simulink model "hopper_6dof_NED_v2_ctv"  (R2025b)
settings: Solver=FixedStepAuto  StartTime=0.0  StopTime=30  FixedStep=1e-3  RelTol=1e-5
values from neighbouring files (symbols this model uses):
  ENGINE = size_engine(IN)    [main_ctv.m]
  fu_mass_profile = linspace(0.1, IN.propulsion.fuel_mass, 200)    [generateBaffleLUT_ctv.m]
  fu_mdot_data = mdot_data(:,2)    [load_lookup_ctv.m]
  g = p.g    [HopperLinearization_6DOF_inertial.m]
  IN = mission_inputs()    [main_ctv.m]
  K1flat = zeros(length(tgrid),52)    [LinerizationMaster_ctv.m]
  K2grid = GainTable.K2'    [LinerizationMaster_ctv.m]
  OUT = Outputs(IN, VEH, TANKS, STRUCT)    [main_ctv.m]
  ox_mass_profile = linspace(0.1, IN.propulsion.oxidizer_mass, 200)    [generateBaffleLUT_ctv.m]
  ox_mdot_data = mdot_data(:,3)    [load_lookup_ctv.m]
  r_leg_1 = [0 IN.legs.feet_radial_dist 0]    [main_ctv.m]
  r_leg_2 = [0 -IN.legs.feet_radial_dist 0]    [main_ctv.m]
  r_leg_3 = [0 0 IN.legs.feet_radial_dist ]    [main_ctv.m]
  r_leg_4 = [0 0 -IN.legs.feet_radial_dist]    [main_ctv.m]
  tank_r = TANKS.singular.radius    [generateBaffleLUT_ctv.m]
  TANKS = size_tanks(IN)    [main_ctv.m]
  Target_Trajectory = [x_trajectory;y_trajectory;z_trajectory;    vx_trajectory;vy_trajectory; vz_trajectory;    P_trajectory; Q_trajectory; R_trajectory ... (first row only)    [LinerizationMaster_ctv.m]
  tgrid = t    [LinerizationMaster_ctv.m]
  thrust_data = mdot_data(:,1)    [load_lookup_ctv.m]
  unom = [T_profile, delta_y_profile, delta_z_profile, rcsp]    [LinerizationMaster_ctv.m]
undefined symbols (not defined in the file or in its folder): cg_init, dcg_dMfu_table, dcg_dMox_table, dI_dMfu_table, dI_dMox_table, engine_cg, engine_mass, fu_axial_damping_ratios, fu_lateral_damping_ratios, fu_masses, MoI_init, mount_cg, ox_axial_damping_ratios, ox_lateral_damping_ratios, ox_masses, pressureLevels, uwndTable, VEH, vwndTable
libraries: fl_lib x31, nesl_utility x25, matrix_library x18, SimscapeFluids_lib x10, simulink_extras x7, slpidlib x7, simulink x7, dspindex x3, aerolibanim x1, commrandsrc3 x1, aerolibutil x1, dspsrcs4 x1
(part 2 of 7)

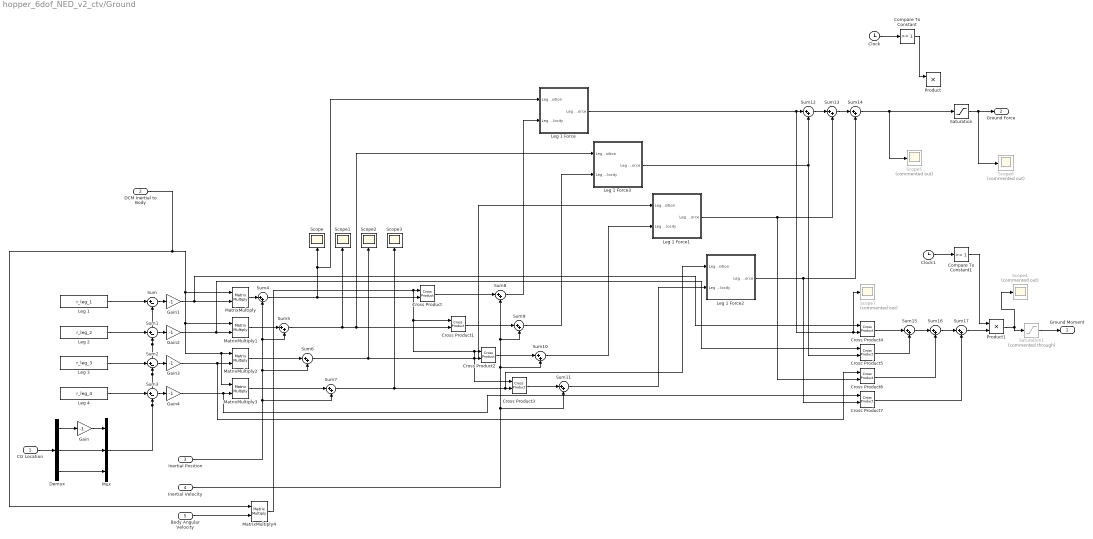
== system hopper_6dof_NED_v2_ctv/Ground  ==
  CG Location : Inport
  DCM Inertial to Body : Inport  Port=2
  Inertial Position : Inport  Port=3
  Inertial Velocity : Inport  Port=4
  Body Angular Velocity : Inport  Port=5
  Clock : Clock
  Clock1 : Clock
  Compare To Constant : simulink/Logic and Bit Operations/Compare To Constant  relop=>=  const=1  OutDataTypeStr=boolean
  Compare To Constant1 : simulink/Logic and Bit Operations/Compare To Constant  relop=>=  const=1  OutDataTypeStr=boolean
  Cross Product{,1..7} (8 alike) : matrix_library/Cross Product
  Demux : Demux  Outputs=3
  Gain{,1..4} (5 alike) : Gain  Gain=-1
  Leg 1 : Constant  Value=r_leg_1
  Leg 1 Force : Subsystem
  Leg 1 Force1 : Subsystem
  Leg 1 Force2 : Subsystem
  Leg 1 Force3 : Subsystem
  Leg 2 : Constant  Value=r_leg_2
  Leg 3 : Constant  Value=r_leg_3
  Leg 4 : Constant  Value=r_leg_4
  MatrixMultiply{,1..4} (5 alike) : Product  Multiplication=Matrix(*)
  Mux : Mux  Inputs=3
  Product : Product
  Product1 : Product
  Saturation : Saturate  UpperLimit=inf  LowerLimit=0
  Saturation1 : Saturate  Commented=through  UpperLimit=inf  LowerLimit=0
  Scope{,1..3} (4 alike) : Scope
      Scope settings: ActiveDisplayYMinimum=-19.811154048207108  ActiveDisplayYMaximum=167.31101950999761  DataLoggingVariableName=ScopeData24
      Scope1 settings: ActiveDisplayYMinimum=182.10765195211306  ActiveDisplayYMaximum=183.93696889205802  DataLoggingVariableName=ScopeData30
      Scope2 settings: DataLoggingVariableName=ScopeData31
      Scope3 settings: DataLoggingVariableName=ScopeData42
  Scope{4..7} (4 alike) : Scope  Commented=on
      Scope4 settings: ActiveDisplayYMinimum=-3.0293963365637429E+7  ActiveDisplayYMaximum=2.2731893212350109E+8  DataLoggingVariableName=ScopeData43
      Scope5 settings: ActiveDisplayYMinimum=-31343.151613259419  ActiveDisplayYMaximum=282088.36451933486  DataLoggingVariableName=ScopeData44
      Scope6 settings: ActiveDisplayYMinimum=-136.62925150266653  ActiveDisplayYMaximum=1229.6632635239991  DataLoggingVariableName=ScopeData45
      Scope7 settings: ActiveDisplayYMinimum=-3.5823523450793636E+8  ActiveDisplayYMaximum=5.8466661508525646E+8  DataLoggingVariableName=ScopeData61
  Sum{,1..3} (4 alike) : Sum  Inputs=|+-
  Sum{4..17} (14 alike) : Sum  Inputs=|++
  Ground Moment : Outport
  Ground Force : Outport  Port=2
  wires:
  Demux/2 -> Mux/2
  Demux/3 -> Mux/3
  Leg 1/1 -> Sum/1
  Leg 2/1 -> Sum1/1
  Leg 3/1 -> Sum2/1
  Leg 4/1 -> Sum3/1
  Mux/1 -> Sum3/2, Sum1/2, Sum/2, Sum2/2
  Sum/1 -> Gain1/1
  DCM Inertial to Body/1 -> MatrixMultiply4/1, MatrixMultiply1/1, MatrixMultiply3/1, MatrixMultiply2/1, MatrixMultiply/1
  Sum1/1 -> Gain2/1
  Sum2/1 -> Gain3/1
  Sum3/1 -> Gain4/1
  MatrixMultiply3/1 -> Sum7/1
  MatrixMultiply2/1 -> Sum6/1
  MatrixMultiply1/1 -> Sum5/1
  MatrixMultiply/1 -> Sum4/1
  Inertial Position/1 -> Sum7/2, Sum6/2, Sum5/2, Sum4/2
  Sum4/1 -> Scope/1, Leg 1 Force/1(Leg Position), Cross Product/2
  Sum5/1 -> Leg 1 Force3/1(Leg Position), Cross Product1/2, Scope1/1
  Sum6/1 -> Leg 1 Force1/1(Leg Position), Cross Product2/2, Scope2/1
  Sum7/1 -> Leg 1 Force2/1(Leg Position), Cross Product3/2, Scope3/1
  Body Angular Velocity/1 -> MatrixMultiply4/2
  MatrixMultiply4/1 -> Cross Product1/1, Cross Product3/1, Cross Product2/1, Cross Product/1
  Cross Product/1 -> Sum8/1
  Cross Product1/1 -> Sum9/1
  Cross Product2/1 -> Sum10/1
  Cross Product3/1 -> Sum11/1
  Inertial Velocity/1 -> Sum11/2, Sum10/2, Sum9/2, Sum8/2
  Leg 1 Force/1(Leg 1 Force) -> Scope7/1, Cross Product4/2, Sum12/1
  Leg 1 Force3/1(Leg 1 Force) -> Cross Product5/2, Sum12/2
  Sum12/1 -> Sum13/1
  Leg 1 Force1/1(Leg 1 Force) -> Cross Product6/2, Sum13/2
  Sum13/1 -> Sum14/1
  Leg 1 Force2/1(Leg 1 Force) -> Cross Product7/2, Sum14/2
  Cross Product4/1 -> Sum15/1
  Sum15/1 -> Sum16/1
  Cross Product5/1 -> Sum15/2
  Cross Product6/1 -> Sum16/2
  Sum16/1 -> Sum17/1
  Cross Product7/1 -> Sum17/2
  Sum8/1 -> Leg 1 Force/2(Leg Velocity)
  Sum9/1 -> Leg 1 Force3/2(Leg Velocity)
  Sum10/1 -> Leg 1 Force1/2(Leg Velocity)
  Sum11/1 -> Leg 1 Force2/2(Leg Velocity)
  Saturation/1 -> Ground Force/1, Scope6/1
  Saturation1/1 -> Ground Moment/1
  Gain/1 -> Mux/1
  Gain1/1 -> Cross Product4/1, MatrixMultiply/2
  Gain2/1 -> Cross Product5/1, MatrixMultiply1/2
  Gain3/1 -> Cross Product6/1, MatrixMultiply2/2
  Gain4/1 -> Cross Product7/1, MatrixMultiply3/2
  Sum14/1 -> Saturation/1, Scope5/1
  Clock1/1 -> Compare To Constant1/1
  Compare To Constant1/1 -> Product1/1
  Sum17/1 -> Product1/2
  Product1/1 -> Scope4/1, Saturation1/1
  CG Location/1 -> Demux/1
  Demux/1 -> Gain/1
  Clock/1 -> Compare To Constant/1
  Compare To Constant/1 -> Product/1

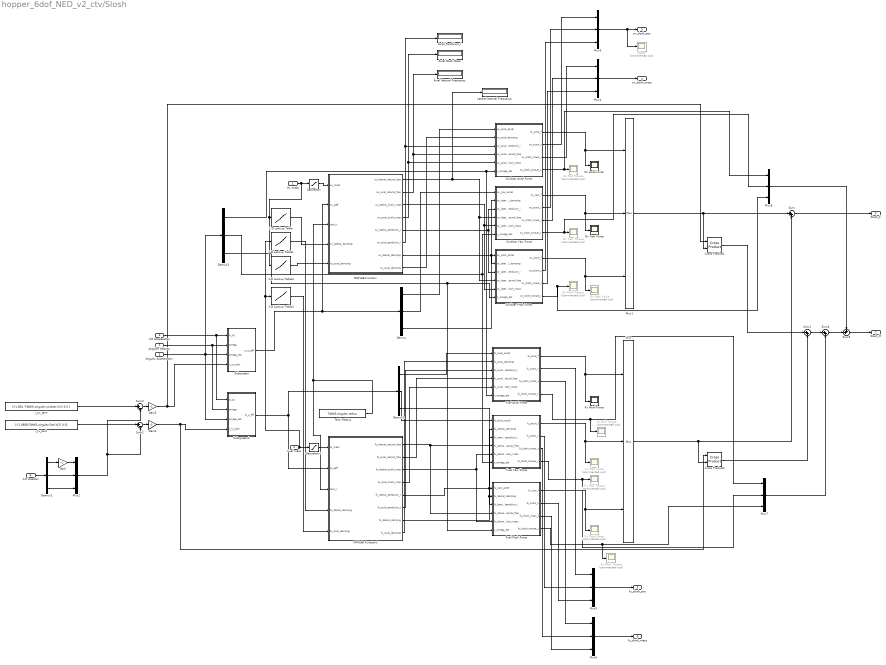
== system hopper_6dof_NED_v2_ctv/Slosh ==
  Ox mass : Inport
  Fuel mass : Inport  Port=2
  CG Acceleration : Inport  Port=3
  Angular Velocity : Inport  Port=4
  Angular Acceleration : Inport  Port=5
  CG Location : Inport  Port=6
  1-D Lookup Table : Lookup_n-D  NumberOfTableDimensions=1  BreakpointsForDimension1=ox_mass_profile  Table=ox_lateral_damping_ratios  InternalRulePriority=Speed  RndMeth=Simplest
  1-D Lookup Table1 : Lookup_n-D  NumberOfTableDimensions=1  BreakpointsForDimension1=fu_mass_profile  Table=fu_lateral_damping_ratios  InternalRulePriority=Speed  RndMeth=Simplest
  1-D Lookup Table2 : Lookup_n-D  NumberOfTableDimensions=1  BreakpointsForDimension1=fu_mass_profile  Table=fu_axial_damping_ratios  InternalRulePriority=Speed  RndMeth=Simplest
  1-D Lookup Table4 : Lookup_n-D  NumberOfTableDimensions=1  BreakpointsForDimension1=ox_mass_profile  Table=ox_axial_damping_ratios  InternalRulePriority=Speed  RndMeth=Simplest
  Axial Natural Frequency : Display
  Axial Slosh Mass : Display
  Axial_Pendulum_l : Display
  Cross Product1 : matrix_library/Cross Product
  Cross Product2 : matrix_library/Cross Product
  Demux{,1..3} (4 alike) : Demux  Outputs=3
  Fu Axial Force : Scope
      settings: ActiveDisplayYMinimum=-4.5487995330933861  ActiveDisplayYMaximum=10.430303988696288  DataLoggingVariableName=ScopeData38
  Fu Pitch Force : Scope  Commented=on
      settings: ActiveDisplayYMinimum=-2.9742058993087932  ActiveDisplayYMaximum=15.331760127930639  DataLoggingVariableName=ScopeData40
  Fu Pitch Torque : Scope  Commented=on
      settings: ActiveDisplayYMinimum=-0.19116574787256713  ActiveDisplayYMaximum=0.19970427620804132  DataLoggingVariableName=ScopeData87
  Fu Roll Torque : Scope  Commented=on
      settings: ActiveDisplayYMinimum=-9.5580450498277436  ActiveDisplayYMaximum=8.6061310713641461  DataLoggingVariableName=ScopeData86
  Fu Yaw Force : Scope  Commented=on
      settings: ActiveDisplayYMinimum=-1.96682346554972  ActiveDisplayYMaximum=2.7427386100438831  DataLoggingVariableName=ScopeData39
  Fu Yaw Torque : Scope  Commented=on
      settings: ActiveDisplayYMinimum=-3.6886267521568623  ActiveDisplayYMaximum=3.9647425854021145  DataLoggingVariableName=ScopeData82
  Fuel Axial Force : Subsystem
  Fuel Pitch Force : Subsystem
  Fuel Yaw Force : Subsystem
  Gain : Gain  Gain=-1
  Gain3 : Gain  Gain=-1
  Gain4 : Gain  Gain=-1
  Lateral Natural Frequency : Display
  MATLAB Function : MATLAB Function  TreatAsAtomicUnit=on
  MATLAB Function1 : MATLAB Function  TreatAsAtomicUnit=on
  Mux{,1..8} (9 alike) : Mux  Inputs=3
  Ox Axial Force : Scope
      settings: ActiveDisplayYMinimum=14.43010515330246  ActiveDisplayYMaximum=16.756383333748122  DataLoggingVariableName=ScopeData34
  Ox Pitch Force : Scope  Commented=on
      settings: ActiveDisplayYMinimum=-4.4950785008236629  ActiveDisplayYMaximum=22.001881619828325  DataLoggingVariableName=ScopeData36
  Ox Pitch Torque : Scope  Commented=on
      settings: ActiveDisplayYMinimum=-0.69593653498138675  ActiveDisplayYMaximum=0.79680864639954685  DataLoggingVariableName=ScopeData85
  Ox Roll Torque : Scope  Commented=on
      settings: ActiveDisplayYMinimum=-0.15656949128956149  ActiveDisplayYMaximum=0.79158034254760723  DataLoggingVariableName=ScopeData80
  Ox Yaw Force : Scope
      settings: ActiveDisplayYMinimum=-5.8284827308381395  ActiveDisplayYMaximum=24.723450598791928  DataLoggingVariableName=ScopeData37
  Ox Yaw Torque : Scope  Commented=on
      settings: ActiveDisplayYMinimum=-0.3482323750211066  ActiveDisplayYMaximum=0.31743853430357161  DataLoggingVariableName=ScopeData81
  Oxidizer Axial Force : Subsystem
  Oxidizer Pitch Force : Subsystem
  Oxidizer Yaw Force : Subsystem
  Saturation : Saturate  UpperLimit=inf  LowerLimit=0.01
  Saturation1 : Saturate  UpperLimit=inf  LowerLimit=0.01
  Scope : Scope  Commented=on
      settings: ActiveDisplayYMinimum=-0.0849364779794028  ActiveDisplayYMaximum=0.368207880424993  DataLoggingVariableName=ScopeData35
  Subsystem : Subsystem
  Subsystem1 : Subsystem
  Sum : Sum  Inputs=|++
  Sum1 : Sum  Inputs=|++
  Sum2 : Sum  Inputs=|+-
  Sum3 : Sum  Inputs=|+-
  Sum4 : Sum  Inputs=|++
  Sum5 : Sum  Inputs=++|
  Tank Radius : Constant  Value=TANKS.singular.radius  SampleTime=-1
  r_fu_tank : Constant  Value=[-(1.0668-TANKS.singular.fuel.h/2) 0 0]
  r_ox_tank : Constant  Value=[-(1.854 -TANKS.singular.oxidizer.h/2) 0 0 ]
  Slosh_F : Outport
  Slosh_M : Outport  Port=2
  ox_slosh_pos : Outport  Port=3
  ox_slosh_mass : Outport  Port=4
  fu_slosh_pos : Outport  Port=5
  fu_slosh_mass : Outport  Port=6
  wires:
  Ox mass/1 -> 1-D Lookup Table4/1, 1-D Lookup Table/1, Saturation/1
  CG Acceleration/1 -> Subsystem/1(a_cg), Subsystem1/1(a_cg)
  Angular Velocity/1 -> Subsystem/2(omega), Subsystem1/2(omega)
  Angular Acceleration/1 -> Subsystem/3(omega_dot), Subsystem1/3(omega_dot), Demux3/1
  Fuel mass/1 -> 1-D Lookup Table2/1, 1-D Lookup Table1/1, Saturation1/1
  Subsystem/1(ox_a_eff) -> Demux/1, MATLAB Function/2(ox_aeff)
  Subsystem1/1(fu_a_eff) -> Demux1/1, MATLAB Function1/2(fu_aeff)
  Demux/1 -> Oxidizer Axial Force/1(ox_axial_accel)
  Demux/2 -> Oxidizer Yaw Force/1(ox_yaw_accel)
  Demux/3 -> Oxidizer Pitch Force/1(ox_pitch_accel)
  Demux1/1 -> Fuel Axial Force/1(fu_axial_accel)
  Demux1/2 -> Fuel Yaw Force/1(fu_pitch_accel)
  Demux1/3 -> Fuel Pitch Force/1(fu_yaw_accel)
  MATLAB Function/1(ox_lateral_natural_freq) -> Lateral Natural Frequency/1, Oxidizer Pitch Force/4(ox_lateral_natural_freq), Oxidizer Yaw Force/4(ox_lateral_natural_freq)
  MATLAB Function/2(ox_axial_natural_freq) -> Axial Natural Frequency/1, Oxidizer Axial Force/4(ox_axial_natural_freq)
  MATLAB Function/3(ox_lateral_slosh_mass) -> Oxidizer Pitch Force/5(ox_lateral_slosh_mass), Oxidizer Yaw Force/5(ox_lateral_slosh_mass)
  MATLAB Function/4(ox_axial_slosh_mass) -> Axial Slosh Mass/1, Oxidizer Axial Force/5(ox_axial_slosh_mass)
  MATLAB Function/5(ox_lateral_pendulum_l) -> Oxidizer Yaw Force/3(ox_lateral_pendulum_l), Oxidizer Pitch Force/3(ox_lateral_pendulum_l)
  MATLAB Function/6(ox_axial_pendulum_l) -> Axial_Pendulum_l/1, Oxidizer Axial Force/3(ox_axial_pendulum_l)
  MATLAB Function/7(ox_lateral_damping) -> Oxidizer Yaw Force/2(ox_lateral_damping), Oxidizer Pitch Force/2(ox_lateral_damping)
  MATLAB Function/8(ox_axial_damping) -> Oxidizer Axial Force/2(ox_axial_damping)
  MATLAB Function1/1(fu_lateral_natural_freq) -> Fuel Pitch Force/4(fu_lateral_natural_freq), Fuel Yaw Force/4(fu_lateral_natural_freq)
  MATLAB Function1/2(fu_axial_natural_freq) -> Fuel Axial Force/4(fu_axial_natural_freq)
  MATLAB Function1/3(fu_lateral_slosh_mass) -> Fuel Yaw Force/5(fu_lateral_slosh_mass), Fuel Pitch Force/5(fu_lateral_slosh_mass)
  MATLAB Function1/4(fu_axial_slosh_mass) -> Fuel Axial Force/5(fu_axial_slosh_mass)
  MATLAB Function1/5(fu_lateral_pendulum_l) -> Fuel Yaw Force/3(fu_lateral_pendulum_l), Fuel Pitch Force/3(fu_lateral_pendulum_l)
  MATLAB Function1/6(fu_axial_pendulum_l) -> Fuel Axial Force/3(fu_axial_pendulum_l)
  MATLAB Function1/7(fu_lateral_damping) -> Fuel Yaw Force/2(fu_lateral_damping), Fuel Pitch Force/2(fu_lateral_damping)
  MATLAB Function1/8(fu_axial_damping) -> Fuel Axial Force/2(fu_axial_damping)
  Fuel Axial Force/1(fu_axial_f) -> Fu Axial Force/1, Mux/1
  Fuel Yaw Force/1(fu_pitch_f) -> Fu Yaw Force/1, Mux/2
  Oxidizer Axial Force/1(ox_axial_f) -> Ox Axial Force/1, Mux1/1
  Oxidizer Yaw Force/1(ox_yaw_f) -> Ox Yaw Force/1, Mux1/2
  Mux1/1 -> Cross Product1/2, Sum/1
  Mux/1 -> Sum/2, Cross Product2/2
  Sum/1 -> Slosh_F/1
  Cross Product1/1 -> Sum1/1
  Cross Product2/1 -> Sum1/2
  Tank Radius/1 -> MATLAB Function1/3(tank_r), MATLAB Function/3(tank_r)
  r_ox_tank/1 -> Sum3/1
  r_fu_tank/1 -> Sum2/1
  Mux2/1 -> Sum2/2, Sum3/2
  Sum3/1 -> Gain3/1
  Sum2/1 -> Gain4/1
  Fuel Pitch Force/1(fu_yaw_f) -> Mux/3, Fu Pitch Force/1
  Oxidizer Pitch Force/1(ox_pitch_f) -> Mux1/3, Ox Pitch Force/1
  Gain3/1 -> Cross Product1/1, Subsystem/4(r_ox_tank)
  Gain4/1 -> Cross Product2/1, Subsystem1/4(r_fu_tank)
  Demux2/3 -> Mux2/3
  CG Location/1 -> Demux2/1
  Demux2/2 -> Mux2/2
  Demux2/1 -> Gain/1
  Gain/1 -> Mux2/1
  Oxidizer Yaw Force/2(ox_slosh_y) -> Mux3/2
  Mux3/1 -> Scope/1, ox_slosh_pos/1
  Oxidizer Axial Force/3(ox_slosh_mass_x) -> Mux4/1
  Oxidizer Yaw Force/3(ox_slosh_mass_y) -> Mux4/2
  Oxidizer Pitch Force/2(ox_slosh_z) -> Mux3/3
  Oxidizer Pitch Force/3(ox_slosh_mass_z) -> Mux4/3
  Mux4/1 -> ox_slosh_mass/1
  Mux5/1 -> fu_slosh_pos/1
  Mux6/1 -> fu_slosh_mass/1
  Fuel Yaw Force/2(fu_slosh_y) -> Mux5/2
  Fuel Pitch Force/2(fu_slosh_z) -> Mux5/3
  Fuel Axial Force/3(fu_slosh_mass_x) -> Mux6/1
  Fuel Yaw Force/3(fu_slosh_mass_y) -> Mux6/2
  Fuel Pitch Force/3(fu_slosh_mass_z) -> Mux6/3
  Oxidizer Axial Force/2(ox_slosh_x) -> Mux3/1
  Fuel Axial Force/2(fu_slosh_x) -> Mux5/1
  Demux3/1 -> Oxidizer Axial Force/6(x_omega_dot), Fuel Axial Force/6(x_omega_dot)
  Demux3/2 -> Fuel Yaw Force/6(y_omega_dot), Oxidizer Yaw Force/6(y_omega_dot)
  Demux3/3 -> Fuel Pitch Force/6(z_omega_dot), Oxidizer Pitch Force/6(z_omega_dot)
  Fuel Axial Force/4(fu_slosh_torque_x) -> Mux7/1, Fu Roll Torque/1
  Fuel Yaw Force/4(fu_slosh_torque_y) -> Mux7/2, Fu Yaw Torque/1
  Fuel Pitch Force/4(fu_slosh_torque_z) -> Mux7/3, Fu Pitch Torque/1
  Oxidizer Axial Force/4(ox_slosh_torque_x) -> Mux8/1, Ox Roll Torque/1
  Oxidizer Pitch Force/4(ox_slosh_torque_z) -> Ox Pitch Torque/1, Mux8/3
  Sum1/1 -> Sum4/1
  Sum5/1 -> Slosh_M/1
  Sum4/1 -> Sum5/2
  Oxidizer Yaw Force/4(ox_slosh_torque_y) -> Mux8/2, Ox Yaw Torque/1
  Mux8/1 -> Sum5/1
  Mux7/1 -> Sum4/2
  Saturation/1 -> MATLAB Function/1(ox_mass)
  Saturation1/1 -> MATLAB Function1/1(fu_mass)
  1-D Lookup Table/1 -> MATLAB Function/4("ox_lateral_damping ")
  1-D Lookup Table1/1 -> MATLAB Function1/4("fu_lateral_damping ")
  1-D Lookup Table4/1 -> MATLAB Function/5("ox_axial_damping ")
  1-D Lookup Table2/1 -> MATLAB Function1/5("fu_axial_damping ")

== system hopper_6dof_NED_v2_ctv/Subsystem ==
  Thrust : Inport
  Fuel mdot : Lookup_n-D  NumberOfTableDimensions=1  BreakpointsForDimension1=thrust_data  Table=fu_mdot_data  InternalRulePriority=Speed  RndMeth=Simplest
  Ox mdot : Lookup_n-D  NumberOfTableDimensions=1  BreakpointsForDimension1=thrust_data  Table=ox_mdot_data  InternalRulePriority=Speed  RndMeth=Simplest
  Fu_mdot : Outport
  Ox_mdot : Outport  Port=2
  wires:
  Thrust/1 -> Ox mdot/1, Fuel mdot/1
  Fuel mdot/1 -> Fu_mdot/1
  Ox mdot/1 -> Ox_mdot/1

== system hopper_6dof_NED_v2_ctv/Subsystem1 ==
  Ox_mdot : Inport
  Fu_mdot : Inport  Port=2
  Integrator : Integrator
  Integrator1 : Integrator
  Ox Mass1 : Constant  Value=IN.propulsion.oxidizer_mass
  Ox Mass2 : Constant  Value=IN.propulsion.fuel_mass
  Saturation : Saturate  UpperLimit=IN.propulsion.oxidizer_mass  LowerLimit=0
  Saturation1 : Saturate  UpperLimit=IN.propulsion.fuel_mass  LowerLimit=0
  Sum : Sum  Inputs=|-+
  Sum1 : Sum  Inputs=|-+
  Ox Mass : Outport
  Fuel Mass : Outport  Port=2
  wires:
  Ox_mdot/1 -> Integrator/1
  Integrator/1 -> Sum/1
  Ox Mass1/1 -> Sum/2
  Sum/1 -> Saturation/1
  Saturation/1 -> Ox Mass/1
  Sum1/1 -> Saturation1/1
  Saturation1/1 -> Fuel Mass/1
  Fu_mdot/1 -> Integrator1/1
  Ox Mass2/1 -> Sum1/2
  Integrator1/1 -> Sum1/1

== system hopper_6dof_NED_v2_ctv/Subsystem2 ==
  Thrust : Inport
  Ox mass : Inport  Port=2
  Fu mass : Inport  Port=3
  If : If  NumInputs=2  IfExpression=u1 > 0 & u2 > 0
  If Action Subsystem : Subsystem  TreatAsAtomicUnit=on
  If Action Subsystem1 : Subsystem  TreatAsAtomicUnit=on
  Merge : Merge
  "Thrust " : Outport
  wires:
  Ox mass/1 -> If/1
  Fu mass/1 -> If/2
  If/1 -> If Action Subsystem/Action
  If/2 -> If Action Subsystem1/Action
  Thrust/1 -> If Action Subsystem1/1(Thrust), If Action Subsystem/1(Thrust)
  If Action Subsystem/1(Out1) -> Merge/1
  If Action Subsystem1/1(Out1) -> Merge/2
  Merge/1 -> "Thrust "/1

== system hopper_6dof_NED_v2_ctv/Subsystem3 ==
  Z : Inport
  W : Inport  Port=2
  Clock : Clock
  Compare To Constant : simulink/Logic and Bit Operations/Compare To Constant  relop=>=  const=5  OutDataTypeStr=boolean
  Constant : Constant
  If : If  NumInputs=2  IfExpression=u1 > -1e-3 & u2 > 0
  If Action Subsystem : Subsystem  TreatAsAtomicUnit=on
  Product : Product
  wires:
  Z/1 -> If/1
  W/1 -> If/2
  If/1 -> If Action Subsystem/Action
  Clock/1 -> Compare To Constant/1
  Compare To Constant/1 -> Product/2
  Constant/1 -> Product/1
  Product/1 -> If Action Subsystem/1(In1)

== system hopper_6dof_NED_v2_ctv/Subsystem4 ==
  Thrust : Inport
  Position : Inport  Port=2
  Velocity : Inport  Port=3
  Demux : Demux  Outputs=3
  Demux1 : Demux  Outputs=3
  If : If  NumInputs=2  IfExpression=u1 > -0.05 & u2 > 0
  If Action Subsystem : Subsystem  TreatAsAtomicUnit=on
  If Action Subsystem1 : Subsystem  TreatAsAtomicUnit=on
  Merge : Merge
  "Thrust " : Outport
  wires:
  If Action Subsystem1/1(Out1) -> Merge/2
  Merge/1 -> "Thrust "/1
  If Action Subsystem/1(Out1) -> Merge/1
  Thrust/1 -> If Action Subsystem1/1(Thrust), If Action Subsystem/1(Thrust)
  Position/1 -> Demux/1
  Demux1/3 -> If/2
  Demux/3 -> If/1
  If/1 -> If Action Subsystem1/Action
  If/2 -> If Action Subsystem/Action
  Velocity/1 -> Demux1/1

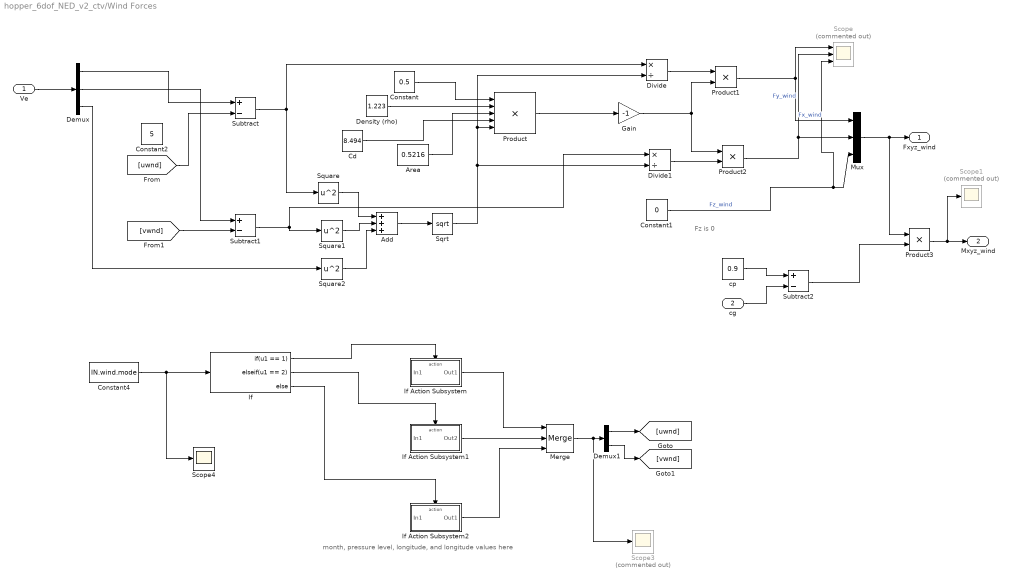
== system hopper_6dof_NED_v2_ctv/Wind Forces ==
  note: month, pressure level, longitude, and longitude values here
  note: Fz is 0
  Ve : Inport
  cg : Inport  Port=2
  Add : Sum  Inputs=+++
  Area : Constant  Value=0.5216
  Cd : Constant  Value=8.494
  Constant : Constant  Value=0.5
  Constant1 : Constant  Value=0
  Constant2 : Constant  Value=5
  Constant4 : Constant  Value=IN.wind.mode
  Demux : Demux  Outputs=3
  Demux1 : Demux  Outputs=2
  Density (rho) : Constant  Value=1.223
  Divide : Product  Inputs=*/
  Divide1 : Product  Inputs=*/
  Gain : Gain  Gain=-1
  If : If  IfExpression=u1 == 1  ElseIfExpressions=u1 == 2
  If Action Subsystem : Subsystem  TreatAsAtomicUnit=on
  If Action Subsystem1 : Subsystem  TreatAsAtomicUnit=on
  If Action Subsystem2 : Subsystem  TreatAsAtomicUnit=on
  Merge : Merge  Inputs=3
  Mux : Mux  Inputs=3
  Product : Product  Inputs=5
  Product1 : Product
  Product2 : Product
  Product3 : Product
  Scope : Scope  Commented=on  NumInputPorts=3
      settings: ActiveDisplayYMinimum=-3.3865408119999993  ActiveDisplayYMaximum=30.478867308  DataLoggingVariableName=ScopeData58
  Scope1 : Scope  Commented=on
      settings: ActiveDisplayYMinimum=-10.256382918668168  ActiveDisplayYMaximum=17.46231209617951  DataLoggingVariableName=ScopeData89
  Scope3 : Scope  Commented=on
      settings: ActiveDisplayYMinimum=4  ActiveDisplayYMaximum=6  DataLoggingVariableName=ScopeData90
  Scope4 : Scope
      settings: ActiveDisplayYMinimum=1  ActiveDisplayYMaximum=3  DataLoggingVariableName=ScopeData91
  Sqrt : Sqrt
  Square : Math  Operator=square
  Square1 : Math  Operator=square
  Square2 : Math  Operator=square
  Subtract : Sum  Inputs=+-
  Subtract1 : Sum  Inputs=+-
  Subtract2 : Sum  Inputs=+-
  cp : Constant  Value=0.9
  Fxyz_wind : Outport
  Mxyz_wind : Outport  Port=2
  wires:
  If/1 -> If Action Subsystem/Action
  Mux/1 -> Product3/1, Fxyz_wind/1
  [vwnd] -> Subtract1/2
  Demux/3 -> Square2/1
  cp/1 -> Subtract2/1
  Divide1/1 -> Product2/2
  Square/1 -> Add/1
  Merge/1 -> Scope3/1, Demux1/1
  Demux1/2 -> [vwnd]
  Product3/1 -> Scope1/1, Mxyz_wind/1
  Gain/1 -> Product1/2, Product2/1
  Subtract2/1 -> Product3/2
  Ve/1 -> Demux/1
  Subtract/1 -> Divide/1, Square/1
  If/2 -> If Action Subsystem1/Action
  Sqrt/1 -> Divide1/2, Divide/2, Product/5
  Demux1/1 -> [uwnd]
  [uwnd] -> Subtract/2
  Area/1 -> Product/3
  Square2/1 -> Add/3
  Product2/1 -> Scope/2, Mux/2  "Fy_wind"
  Constant4/1 -> Scope4/1, If/1
  Constant1/1 -> Scope/3, Mux/3  "Fz_wind"
  If/3 -> If Action Subsystem2/Action
  Product1/1 -> Scope/1, Mux/1  "Fx_wind"
  Cd/1 -> Product/4
  Subtract1/1 -> Square1/1, Divide1/1
  Density (rho)/1 -> Product/2
  If Action Subsystem/1(Out1) -> Merge/1
  cg/1 -> Subtract2/2
  If Action Subsystem2/1(Out1) -> Merge/3
  Constant/1 -> Product/1
  Demux/2 -> Subtract1/1
  If Action Subsystem1/1(Out2) -> Merge/2
  Divide/1 -> Product1/1
  Add/1 -> Sqrt/1
  Product/1 -> Gain/1
  Square1/1 -> Add/2
  Demux/1 -> Subtract/1

== system hopper_6dof_NED_v2_ctv/Control Inputs -> Fxyz & Mxyz/EDF Dynamics ==
  Cmd Torque : Inport
  Divide : Product  Inputs=*/
  Product : Product
  Product1 : Product
  Quantizer2 : Quantizer  QuantizationInterval=IN.rcs.resolution
  Radius : Constant  Value=TANKS.singular.radius
  Rate Limiter : RateLimiter  RisingSlewLimit=25  FallingSlewLimit=-25  SampleTimeMode=inherited
  Saturation : Saturate  Commented=through  UpperLimit=1  LowerLimit=0  ZeroCross=off
  Saturation1 : Saturate  UpperLimit=IN.rcs.max_thrust  LowerLimit=-IN.rcs.max_thrust  ZeroCross=off
  Transfer Fcn : TransferFcn  Denominator=[IN.rcs_time_constant 1]
  max Thrust : Constant  Value=IN.rcs.max_thrust
  "Real Torque " : Outport
  wires:
  Divide/1 -> Saturation/1
  Radius/1 -> Product/2
  Product/1 -> Product1/2, Divide/2
  Cmd Torque/1 -> Divide/1
  max Thrust/1 -> Product/1
  Transfer Fcn/1 -> Product1/1
  Product1/1 -> Quantizer2/1
  Saturation/1 -> Transfer Fcn/1
  Quantizer2/1 -> Rate Limiter/1
  Rate Limiter/1 -> Saturation1/1
  Saturation1/1 -> "Real Torque "/1
